simulink model "SIMULINK_Fuzzy"  (R2023b)
settings: Solver=ode23tb  StartTime=0.0  StopTime=10000  MaxStep=1  RelTol=1e-5  AbsTol=1e-7
model workspace (MAT data in the model file):
  Cth = 40.5
  Idis_plot = 0.95652
  Ilimit = 2.2
  Qrated = 2.2
  R0 = 0.016818
  Rth = 20
  SOC0 = [2.5 2.5 2.5 2.5]
  SOCstop = 99
  StopAtVoltage = 1
  Tamb = 25
  Tresponse = 10
  TsFIS = 1
  TsPower = 1
  Vcutoff = 4.2
  Vnom = 3.7
undefined symbols (not defined in the file or in its folder): Ion, Lithium
libraries: spsBatteryLib x4, fuzblock x2, simulink x2, spsControlledCurrentSourceLib x1, spsCurrentMeasurementLib x1, spsVoltageMeasurementLib x1, sps_lib x1
settings Model: Creator=LeoNick  LastModifiedBy=Leo Nick
settings DataIOCC: SaveOutput=off

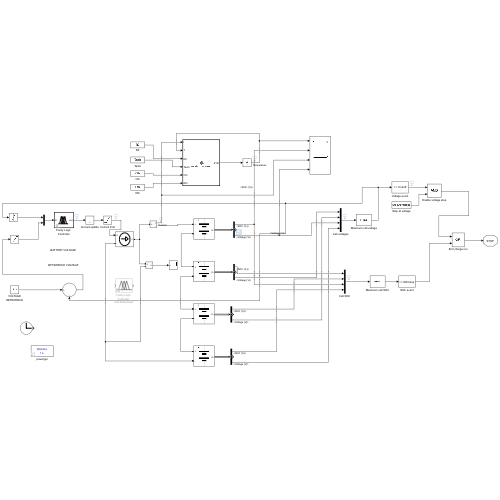
[thumbnail: Simulink's stored preview of the top-level diagram]
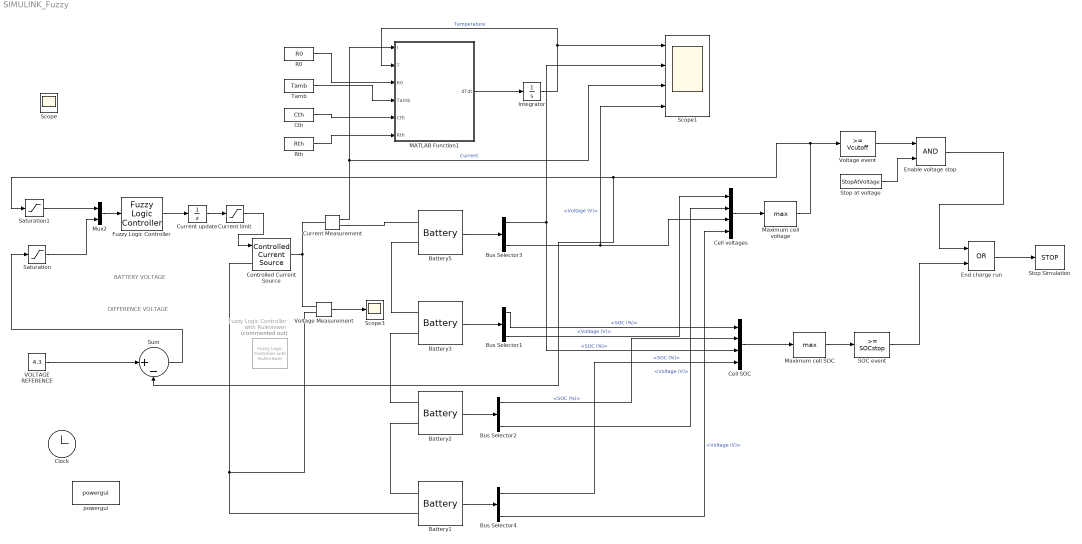
== system SIMULINK_Fuzzy ==
  note: BATTERY VOLTAGE
  note: DIFFERENCE VOLTAGE
  Battery1 : spsBatteryLib/Battery  BatType=Lithium-Ion  ShowTempParam=off  ThermalPreset=no  ShowAgeParam=off  NomV=Vnom  NomQ=Qrated  SOC=SOC0(4)  Batt_Tr=Tresponse  PresetModel=on  MaxQ=2.2  MinV=2.775  FullV=4.3068  Dis_rate=0.95652  R=0.016818  Normal_OP=1.9896  expZone="[3.9974     0.10809]"  current=Idis_plot  Units=Time  Tci=20  NomT=20  T2=-30  MaxQ2=4.8  FullV2=7.1  Normal_OP2=5.655  expZone2="[6.58           1]"  Rca=0.6  ti=2000  Dp=0  Neq0=0  Tsim=1e6  Ta1=25  Qeol=5.4*0.9  Reol=0.013333*1.2  Char_age=[2.3478, 3]  Dis_age=[2.3478, 10]  N1=1500  N2=10500  N3=1000  N4=1400  Ta2=45  N5=950
  Battery2 : spsBatteryLib/Battery  BatType=Lithium-Ion  ShowTempParam=off  ThermalPreset=no  ShowAgeParam=off  NomV=Vnom  NomQ=Qrated  SOC=SOC0(2)  Batt_Tr=Tresponse  PresetModel=on  MaxQ=2.2  MinV=2.775  FullV=4.3068  Dis_rate=0.95652  R=0.016818  Normal_OP=1.9896  expZone="[3.9974     0.10809]"  current=Idis_plot  Units=Time  Tci=20  NomT=20  T2=-30  MaxQ2=4.8  FullV2=7.1  Normal_OP2=5.655  expZone2="[6.58           1]"  Rca=0.6  ti=2000  Dp=0  Neq0=0  Tsim=1e6  Ta1=25  Qeol=5.4*0.9  Reol=0.013333*1.2  Char_age=[2.3478, 3]  Dis_age=[2.3478, 10]  N1=1500  N2=10500  N3=1000  N4=1400  Ta2=45  N5=950
  Battery3 : spsBatteryLib/Battery  BatType=Lithium-Ion  ShowTempParam=off  ThermalPreset=no  ShowAgeParam=off  NomV=Vnom  NomQ=Qrated  SOC=SOC0(1)  Batt_Tr=Tresponse  PresetModel=on  MaxQ=2.2  MinV=2.775  FullV=4.3068  Dis_rate=0.95652  R=0.016818  Normal_OP=1.9896  expZone="[3.9974     0.10809]"  current=Idis_plot  Units=Time  Tci=20  NomT=20  T2=-30  MaxQ2=4.8  FullV2=7.1  Normal_OP2=5.655  expZone2="[6.58           1]"  Rca=0.6  ti=2000  Dp=0  Neq0=0  Tsim=1e6  Ta1=25  Qeol=5.4*0.9  Reol=0.013333*1.2  Char_age=[2.3478, 3]  Dis_age=[2.3478, 10]  N1=1500  N2=10500  N3=1000  N4=1400  Ta2=45  N5=950
  Battery5 : spsBatteryLib/Battery  BatType=Lithium-Ion  ShowTempParam=off  ThermalPreset=no  ShowAgeParam=off  NomV=Vnom  NomQ=Qrated  SOC=SOC0(3)  Batt_Tr=Tresponse  PresetModel=on  MaxQ=2.2  MinV=2.775  FullV=4.3068  Dis_rate=0.95652  R=0.016818  Normal_OP=1.9896  expZone="[3.9974     0.10809]"  current=Idis_plot  Units=Time  Tci=20  NomT=20  T2=-30  MaxQ2=4.8  FullV2=7.1  Normal_OP2=5.655  expZone2="[6.58           1]"  Rca=0.6  ti=2000  Dp=0  Neq0=0  Tsim=1e6  Ta1=25  Qeol=5.4*0.9  Reol=0.013333*1.2  Char_age=[2.3478, 3]  Dis_age=[2.3478, 10]  N1=1500  N2=10500  N3=1000  N4=1400  Ta2=45  N5=950
  Bus Selector{1..4} (4 alike) : BusSelector  OutputSignals=SOC (%),Current (A),Voltage (V)
  Cell SOC : Mux
  Cell voltages : Mux
  Clock : Clock
  Controlled Current Source : spsControlledCurrentSourceLib/Controlled Current Source  Initialize=on  Source_Type=DC  Amplitude=0  Phase=0  Frequency=0  Measurements=None
  Cth : Constant  Value=Cth
  Current Measurement : spsCurrentMeasurementLib/Current Measurement  PhasorSimulation=off  OutputType=Complex  PSBequivalent=0
  Current limit : Saturate  UpperLimit=Ilimit  LowerLimit=0
  Current update : UnitDelay  SampleTime=TsFIS  HasFrameUpgradeWarning=on
  Enable voltage stop : Logic  AllPortsSameDT=off  OutDataTypeStr=boolean
  End charge run : Logic  Operator=OR  AllPortsSameDT=off  OutDataTypeStr=boolean
  Fuzzy Logic Controller : fuzblock/Fuzzy Logic  Controller  FIS='Fuzzy_2_2A.fis'  OutputSampleNumber=101  DataType=double  FuzzifiedInputs=off  RuleFiringStrengths=off  RuleOutputs=off  AggregatedOutputs=off  SimulateUsing=Interpreted execution  OutOfRangeInputValueMessage=warning  NoRuleFiredMessage=warning  EmptyOutputFuzzySetMessage=warning
  Fuzzy Logic Controller with Ruleviewer : fuzblock/Fuzzy Logic  Controller  with Ruleviewer  Commented=on  fismatrix=fisrule  Ts=1
  Integrator : Integrator  InitialCondition=Tamb
  MATLAB Function1 : MATLAB Function  TreatAsAtomicUnit=on
  Maximum cell SOC : MinMax  Function=max
  Maximum cell voltage : MinMax  Function=max
  Mux2 : Mux  Inputs=2
  R0 : Constant  Value=R0
  Rth : Constant  Value=Rth
  SOC event : simulink/Logic and Bit Operations/Compare To Constant  relop=>=  const=SOCstop  OutDataTypeStr=boolean
  Saturation : Saturate  UpperLimit=1.22  LowerLimit=0
  Saturation1 : Saturate  UpperLimit=4.3  LowerLimit=3.08
  Scope1 : Scope  NumInputPorts=4
  Scope3 : Scope
  Stop Simulation : Stop
  Stop at voltage : Constant  Value=StopAtVoltage
  Sum : Sum  Inputs=|+-
  Tamb : Constant  Value=Tamb
  VOLTAGE REFERENCE : Constant  Value=4.3
  Voltage Measurement : spsVoltageMeasurementLib/Voltage Measurement  PhasorSimulation=off  OutputType=Complex  PSBequivalent=0
  Voltage event : simulink/Logic and Bit Operations/Compare To Constant  relop=>=  const=Vcutoff  OutDataTypeStr=boolean
  powergui : sps_lib/powergui  Priority=1  SimulationMode=Discrete  SampleTime=TsPower  frequency=60  Iterations=50  frequencyindice=0  Pbase=100e6  ErrMax=1e-4  UnitsV=kV  UnitsW=MW  buscounter=0  FunctionMessages=off  echomessages=off  EnableUseOfTLC=off  CurrentSourceSwitches=off  DisableSnubberDevices=off  DisableRonSwitches=off  DisableVfSwitches=off  DisplayEquations=off  AutomaticDiscreteSolvers=off  SolverType=Tustin/Backward Euler (TBE)  Interpol=off  ExternalGateDelay=off  methode=off  Ts=100  x0status=blocks  SPID=on  SwTol=0  HookPort=off  NonlinearTolerance=1e-4  nMaxIteration=100  ContinueOnMaxIteration=off  RestoreLinks=warning  ResistiveCurrentMeasurement=off  Frange=[0:2:500]  Ylog=off  Xlog=on  ShowGrid=off  save=off  variable=ZData  structure=0  ZoomFFT=off  StartTime=0.0  cycles=1  DisplayStyle=1  fundamental=60  FreqAxis=off  MaxFrequency=1000  frequencyindicesteady=1  RmsSteady=1  display=off
  Scope : Scope
  wires:
  Voltage Measurement/1 -> Scope3/1
  VOLTAGE REFERENCE/1 -> Sum/1
  Sum/1 -> Saturation/1
  Current update/1 -> Current limit/1
  Saturation/1 -> Mux2/2
  Saturation1/1 -> Mux2/1
  Battery3/1 -> Bus Selector1/1
  Bus Selector4/1 -> Cell SOC/4  "<SOC (%)>"
  Bus Selector4/3 -> Cell voltages/4  "<Voltage (V)>"
  Bus Selector2/1 -> Cell SOC/2  "<SOC (%)>"
  Battery1/1 -> Bus Selector4/1
  Bus Selector3/1 -> Scope1/2, Cell SOC/3  "<SOC (%)>"
  Bus Selector1/3 -> Cell voltages/1  "<Voltage (V)>"
  Bus Selector2/3 -> Cell voltages/2  "<Voltage (V)>"
  Bus Selector3/3 -> Cell voltages/3, Scope1/4  "<Voltage (V)>"
  Bus Selector1/1 -> Cell SOC/1  "<SOC (%)>"
  Battery5/1 -> Bus Selector3/1
  Battery2/1 -> Bus Selector2/1
  Mux2/1 -> Fuzzy Logic Controller/1
  Current Measurement/1 -> Scope1/3, MATLAB Function1/1(I)  "Current"
  Integrator/1 -> Scope1/1, MATLAB Function1/2(T)  "Temperature"
  MATLAB Function1/1(dTdt) -> Integrator/1
  Fuzzy Logic Controller/1 -> Current update/1
  Current limit/1 -> Controlled Current Source/1
  Cell voltages/1 -> Maximum cell voltage/1
  Cell SOC/1 -> Maximum cell SOC/1
  Maximum cell voltage/1 -> Sum/2, Saturation1/1, Voltage event/1
  Maximum cell SOC/1 -> SOC event/1
  Voltage event/1 -> Enable voltage stop/1
  Stop at voltage/1 -> Enable voltage stop/2
  Enable voltage stop/1 -> End charge run/1
  SOC event/1 -> End charge run/2
  End charge run/1 -> Stop Simulation/1
  R0/1 -> MATLAB Function1/3(R0)
  Tamb/1 -> MATLAB Function1/4(Tamb)
  Cth/1 -> MATLAB Function1/5(Cth)
  Rth/1 -> MATLAB Function1/6(Rth)
  connections:
  Controlled Current Source/LConn1 -- Battery1/LConn2 -- Voltage Measurement/LConn2
  Controlled Current Source/RConn1 -- Current Measurement/LConn1 -- Voltage Measurement/LConn1
  Battery1/LConn1 -- Battery2/LConn2
  Battery3/LConn2 -- Battery2/LConn1
  Battery5/LConn2 -- Battery3/LConn1
  Current Measurement/RConn1 -- Battery5/LConn1

== matlab function SIMULINK_Fuzzy/MATLAB Function1 ==
  data: I input; dTdt output; T input; R0 input; Tamb input; Cth input; Rth input
function dTdt = modelo_termico(I,T,R0,Tamb,Cth,Rth)
dTdt = (I^2*R0 - (T-Tamb)/Rth)/Cth;
end
